simulink model "ladrc_model_2nd"  (R2024a)
settings: Solver=ode4  StartTime=0.0  StopTime=10.0  FixedStep=0.001  RelTol=1e-3
values from neighbouring files (symbols this model uses):
  K = 1    [Q1_a_1.m]    (also in Q1_a_2.m; Q1_a_3.m; Q1_a_4.m; Q1_a_5.m)
  k_ob_const = 10    [Q1_a_6.m]
  T = T_values(i)    [Q1_a_1.m]    (also in Q1_a_2.m = T_values(ti); Q1_a_3.m = T_values(ti); Q1_a_4.m = 1; Q1_a_5.m = 1)
  T_dead = 0    [Q1_a_6.m]
  T_dead_ESO = 0    [Q1_a_6.m]
undefined symbols (not defined in the file or in its folder): D, Ki_pi, Kp_pi
libraries: slpidlib x1
settings Model: Creator=Asus  LastModifiedBy=Asus

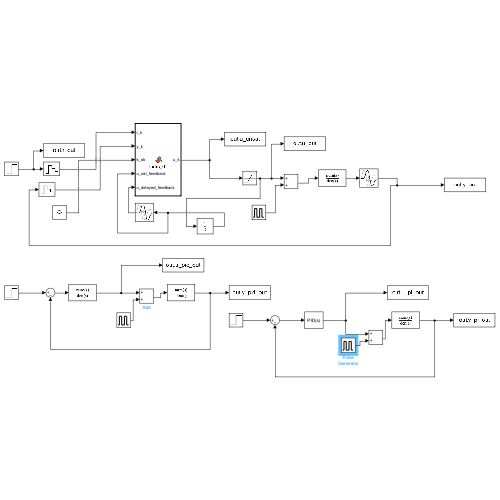
[thumbnail: Simulink's stored preview of the top-level diagram]
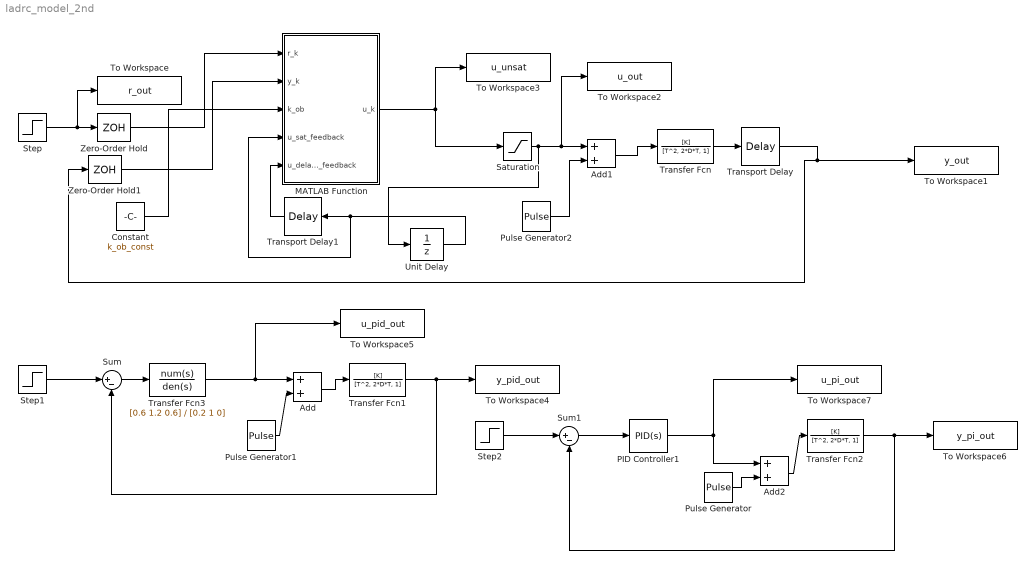
== system ladrc_model_2nd ==
  Add : Sum
  Add1 : Sum
  Add2 : Sum
  Constant : Constant  Value=k_ob_const  SampleTime=0.001
  MATLAB Function : MATLAB Function  TreatAsAtomicUnit=on  SystemSampleTime=0.001
  PID Controller1 : slpidlib/PID Controller  Controller=PID  Form=Parallel  TimeDomain=Continuous-time  UseExternalTs=off  SampleTime=-1  IntegratorMethod=Forward Euler  FilterMethod=Forward Euler  ControllerParametersSource=internal  P=Kp_pi  I=Ki_pi  UseKiTs=off  D=0  UseExternalDerivativeSource=off  N=100  UseFilter=on  TunerSelectOption=Transfer Function Based (PID Tuner App)  InitialConditionSource=internal  InitialConditionForIntegrator=0  InitialConditionForFilter=0  DifferentiatorICPrevScaledInput=0  ExternalReset=none  TrackingMode=off  Kt=1  LimitOutput=off  SatLimitsSource=internal  UpperSaturationLimit=inf  LowerSaturationLimit=-inf  LinearizeAsGain=on  AntiWindupMode=none  Kb=1  LimitIntegrator=off  UpperIntegratorSaturationLimit=inf  LowerIntegratorSaturationLimit=-inf  POutMin=[]  POutMax=[]  IOutMin=[]  IOutMax=[]  DOutMin=[]  DOutMax=[]  NOutMin=[]  NOutMax=[]  SumOutMin=[]  SumOutMax=[]  SaturationOutMin=[]  SaturationOutMax=[]  PParamMin=[]  PParamMax=[]  IParamMin=[]  IParamMax=[]  DParamMin=[]  DParamMax=[]  NParamMin=[]  NParamMax=[]  KbParamMin=[]  KbParamMax=[]  KtParamMin=[]  KtParamMax=[]  KbOutMin=[]  KbOutMax=[]  KtOutMin=[]  KtOutMax=[]  IntegratorOutMin=[]  IntegratorOutMax=[]  FilterOutMin=[]  FilterOutMax=[]  SumI1OutMin=[]  SumI1OutMax=[]  SumI2OutMin=[]  SumI2OutMax=[]  SumI3OutMin=[]  SumI3OutMax=[]  SumI4OutMin=[]  SumI4OutMax=[]  SumDOutMin=[]  SumDOutMax=[]  DifferentiatorOutMin=[]  DifferentiatorOutMax=[]  FilterDiffOutCoefMin=[]  FilterDiffOutCoefMax=[]  ReciprocalOutMin=[]  ReciprocalOutMax=[]  SumDenOutMin=[]  SumDenOutMax=[]  SumNumOutMin=[]  SumNumOutMax=[]  DivideOutMin=[]  DivideOutMax=[]  UdiffTsProdOutMin=[]  UdiffTsProdOutMax=[]  NTsProdOutMin=[]  NTsProdOutMax=[]  UintegralTsProdOutMin=[]  UintegralTsProdOutMax=[]  UngainTsProdOutMin=[]  UngainTsProdOutMax=[]  ClampingZeroOutDataTypeStr=Inherit: Inherit via back propagation  ClampingZeroOutMin=[]  ClampingZeroOutMax=[]  FilterDenConstantOutDataTypeStr=Inherit: Inherit via back propagation  FilterDenConstantOutMin=[]  FilterDenConstantOutMax=[]  PCopyOutDataTypeStr=Inherit: Inherit via back propagation  PCopyOutMin=[]  PCopyOutMax=[]  NCopyOutDataTypeStr=Inherit: Inherit via back propagation  NCopyOutMin=[]  NCopyOutMax=[]  IntegratorContinuousStateAttributes=''  IntegratorStateMustResolveToSignalObject=off  IntegratorRTWStateStorageClass=Auto  FilterContinuousStateAttributes=''  FilterStateMustResolveToSignalObject=off  FilterRTWStateStorageClass=Auto  ParallelPVariant=InternalParameters  IdealPVariant=Disabled  IVariant=InternalParameters  DVariant=InternalParameters  IntegratorVariant=Continuous  SatVariant=Disabled  AWVariant=Passthrough  PCopyVariant=Disabled  TRVariant=Disabled  FdbkBlocksVariant=Forward  IdealPFdbkVariant=Disabled  SatFdbkVariant=Disabled  DerivativeFilterVariant=ContFilter  NVariant=InternalParameters  NCopyVariant=Disabled  FilterICVariant=InternalICsFilter  IntegratorICVariant=InternalICs  ExternalResetVariant=Disabled  TRSumVariant=Passthrough  SumFdbkVariant=Disabled  SumVariant=Sum_PID  TsampFilterVariant=InternalTs  TsampNgainVariant=Passthrough  TsampIntegralVariant=Disabled_SignalSpec  ExternalSaturationOutDataTypeStr=Inherit: Same as second input  DerivativeSourceVariant=ErrorSignal
  Pulse Generator : DiscretePulseGenerator  PulseType=Time based  Amplitude=0.5  Period=40  PulseWidth=25  PhaseDelay=15
  Pulse Generator1 : DiscretePulseGenerator  PulseType=Time based  Amplitude=0.5  Period=40  PulseWidth=25  PhaseDelay=15
  Pulse Generator2 : DiscretePulseGenerator  PulseType=Time based  Amplitude=0.5  Period=40  PulseWidth=25  PhaseDelay=15
  Saturation : Saturate  UpperLimit=100  LowerLimit=-100
  Step : Step  Time=0  SampleTime=0
  Step1 : Step  Time=0  SampleTime=0
  Step2 : Step  Time=0  SampleTime=0
  Sum : Sum  Inputs=|+-
  Sum1 : Sum  Inputs=|+-
  To Workspace : ToWorkspace  VariableName=r_out  SampleTime=-1
  To Workspace1 : ToWorkspace  VariableName=y_out  SampleTime=-1
  To Workspace2 : ToWorkspace  VariableName=u_out  SampleTime=-1
  To Workspace3 : ToWorkspace  VariableName=u_unsat  SampleTime=0.001
  To Workspace4 : ToWorkspace  VariableName=y_pid_out  SampleTime=0.001
  To Workspace5 : ToWorkspace  VariableName=u_pid_out  SampleTime=-1
  To Workspace6 : ToWorkspace  VariableName=y_pi_out  SampleTime=0.001
  To Workspace7 : ToWorkspace  VariableName=u_pi_out  SampleTime=-1
  Transfer Fcn : TransferFcn  Numerator=[K]  Denominator=[T^2, 2*D*T, 1]
  Transfer Fcn1 : TransferFcn  Numerator=[K]  Denominator=[T^2, 2*D*T, 1]
  Transfer Fcn2 : TransferFcn  Numerator=[K]  Denominator=[T^2, 2*D*T, 1]
  Transfer Fcn3 : TransferFcn  Numerator=[0.6 1.2 0.6]  Denominator=[0.2 1 0]
  Transport Delay : TransportDelay  DelayTime=T_dead
  Transport Delay1 : TransportDelay  DelayTime=T_dead_ESO
  Unit Delay : UnitDelay  SampleTime=0.001  HasFrameUpgradeWarning=on
  Zero-Order Hold : ZeroOrderHold  SampleTime=-1
  Zero-Order Hold1 : ZeroOrderHold  SampleTime=-1
  wires:
  MATLAB Function/1(u_k) -> Saturation/1, To Workspace3/1
  Step/1 -> To Workspace/1, Zero-Order Hold/1
  Zero-Order Hold/1 -> MATLAB Function/1(r_k)
  Zero-Order Hold1/1 -> MATLAB Function/2(y_k)
  Constant/1 -> MATLAB Function/3(k_ob)
  Unit Delay/1 -> MATLAB Function/4(u_sat_feedback), Transport Delay1/1
  Transport Delay/1 -> Zero-Order Hold1/1, To Workspace1/1
  Transport Delay1/1 -> MATLAB Function/5(u_delayed_feedback)
  Transfer Fcn/1 -> Transport Delay/1
  Step1/1 -> Sum/1
  Transfer Fcn1/1 -> To Workspace4/1, Sum/2
  Saturation/1 -> Unit Delay/1, Add1/1, To Workspace2/1
  Transfer Fcn3/1 -> Add/1, To Workspace5/1
  Sum1/1 -> PID Controller1/1
  Step2/1 -> Sum1/1
  Transfer Fcn2/1 -> To Workspace6/1, Sum1/2
  PID Controller1/1 -> To Workspace7/1, Add2/1
  Sum/1 -> Transfer Fcn3/1
  Pulse Generator1/1 -> Add/2
  Add/1 -> Transfer Fcn1/1
  Pulse Generator/1 -> Add2/2
  Add2/1 -> Transfer Fcn2/1
  Pulse Generator2/1 -> Add1/2
  Add1/1 -> Transfer Fcn/1

== matlab function ladrc_model_2nd/MATLAB Function ==
  data: r_k input; u_k output; y_k input; k_ob input; u_sat_feedback input; u_delayed_feedback input
function u_k = ladrc_dt(r_k, y_k, k_ob, u_sat_feedback, u_delayed_feedback)
    % tuning parameters, im writing the code for this block as following so
    % i only have to change these paramters every time
    T_settle = 5;
    b0 = 1;
    Ts = 0.001;

    % persistent variables holding states from step (k-1)
    persistent x_hat_k_minus_1 u_k_minus_1
    if isempty(x_hat_k_minus_1)
        x_hat_k_minus_1 = [0; 0; 0];
        u_k_minus_1 = 0;
    end

    % kp, kd, poles, L, Ad, Bd, Cd
    s_CL = -6 / T_settle;
    Kp   = s_CL^2;
    Kd   = -2 * s_CL;

    % ESO poles all at s_ESO
    s_ESO = k_ob * s_CL;
    z_ESO = exp(s_ESO * Ts);

    % 3rd order ESO gains from slide eq(43)
    l1 = 1 - z_ESO^3;
    l2 = (3 / (2*Ts))  * (1 - z_ESO)^2 * (1 + z_ESO);
    l3 = (1 / Ts^2)    * (1 - z_ESO)^3;
    Ld = [l1; l2; l3];

    % Ad, Bd, Cd from slide eq(35)
    Ad = [1,  Ts,  Ts^2/2;
          0,   1,  Ts;
          0,   0,  1];
    Bd = [b0*Ts^2/2;
          b0*Ts;
          0];
    Cd = [1, 0, 0];

    % observer would calculate current estimate x_hat(k)
    x_hat_k = (Ad - Ld*Cd*Ad) * x_hat_k_minus_1 + (Bd - Ld*Cd*Bd) * u_k_minus_1 + Ld * y_k;

    % our control Law would calculate current output u(k)
    u_k = (1/b0) * (Kp*(r_k - x_hat_k(1)) - Kd*x_hat_k(2) - x_hat_k(3));

    % update Memory for next Step (Current becomes k-1 for the next loop)
    x_hat_k_minus_1 = x_hat_k;
    u_k_minus_1 = u_delayed_feedback;
end
